simulink model "ASM_Traffic_new"  (R2024a)
settings: Solver=ode1  StartTime=SIM.tstart.v  StopTime=SIM.tend.v  FixedStep=SIM.StepSize.v  RelTol=1e-3
PostLoadFcn:
  | if any(exist('dsrtsu_mdlpostloadfcn', 'file') ~= 0), dsrtsu_mdlpostloadfcn('Execute', bdroot); end
  | try, asm_mdl_postloadfcn(bdroot, 'UpdateModel', 3600); catch, disp(lasterr); end,
InitFcn:
  | , if any(exist('rtifpga_mdlclblib', 'file') ~= 0), rtifpga_mdlclblib('Init', bdroot); end,
  | , if any(exist('dsmpb_private', 'file') ~= 0), dsmpb_private('dsmpb_mdlclblib', 'Init', bdroot); end,
undefined symbols (not defined in the file): _to_, a0b2, ASM_BrakeHydraulics_DemoSystems, ASM_VehicleDynamics_DemoSystems, b98103fe8ad365046cd0, BrakeCircuit, CPT, Crankshaft, DiscIntNeverNeededParam, dsmsi, FinalDriveAssembly, MDL, ModeSignals, Pos_BrakePedal_Maneuver, rad, RefSignals, s_to_rpm, SIM, SoftECU, Suspension, Tire, Transmission
libraries: ASM_Traffic_lib x135, simulink x100, ASM_Utils_lib x77, ASM_VehicleDynamics_lib x70, ASM_Environment_lib x22, dsmpblib x20, dsmsilib x15, MDLD_Utils_lib x10, ASM_BrakeHydraulics_lib x3
(part 12 of 63)

== system ASM_Traffic_new/Engine/Interface_Out/Control_ModelSignals ==
  State_ICEngine[0|1|2|3|4] : Inport
  n_Engine_Idle_Set[rpm] : Inport  Port=2
  Sw_Starter[0Off|1On] : Inport  Port=3
  Enable_Trq_Shift_Request[0|1] : Inport  Port=4
  Trq_Shift_Request[Nm] : Inport  Port=5
  State_StartStop[1Off|2NotReady|3Ready|4EngStopped] : Inport  Port=6
  CrankAngle_Cyl[aTDC] : Inport  Port=7
  p_Ambient[Pa] : Inport  Port=8
  T_Ambient[degC] : Inport  Port=9
  Sw_Replace_Env[0|1] : Inport  Port=10
  EngOP_Num[] : Inport  Port=11
  Pos_AccPedal_Meas[%] : Inport  Port=12
  n_Engine_Meas[rpm] : Inport  Port=13
  Trq_MeanEff_Engine_Meas[Nm] : Inport  Port=14
  Bus Creator : BusCreator  Inputs=14
  CrankAngle_Cyl[aTDC]_ : Subsystem
      mask Display: disp('')
  Enable_Trq_Shift_Request[0|1]_ : Subsystem
      mask Display: disp('')
  EngOP_Num[]_ : Subsystem
      mask Display: disp('')
  Pos_AccPedal_Meas[%]_ : Subsystem
      mask Display: disp('')
  State_ICEngine[0|1|2|3|4]_ : Subsystem
      mask Display: disp('')
  State_StartStop[1Off|2NotReady|3Ready|4EngStopped]_ : Subsystem
      mask Display: disp('')
  Sw_Replace_Env[0|1]_ : Subsystem
      mask Display: disp('')
  Sw_Starter[0Off|1On]_ : Subsystem
      mask Display: disp('')
  T_Ambient[degC]_ : Subsystem
      mask Display: disp('')
  Trq_MeanEff_Engine_Meas[Nm]_ : Subsystem
      mask Display: disp('')
  Trq_Shift_Request[Nm]_ : Subsystem
      mask Display: disp('')
  n_Engine_Idle_Set[rpm]_ : Subsystem
      mask Display: disp('')
  n_Engine_Meas[rpm]_ : Subsystem
      mask Display: disp('')
  p_Ambient[Pa]_ : Subsystem
      mask Display: disp('')
  Out : Outport  VectorParamsAs1DForOutWhenUnconnected=off
  wires:
  T_Ambient[degC]_/1(Out1) -> Bus Creator/9  "T_Ambient[degC]"
  p_Ambient[Pa]_/1(Out1) -> Bus Creator/8  "p_Ambient[Pa]"
  CrankAngle_Cyl[aTDC]_/1(Out1) -> Bus Creator/7  "CrankAngle_Cyl[aTDC]"
  T_Ambient[degC]/1 -> T_Ambient[degC]_/1(In1)
  p_Ambient[Pa]/1 -> p_Ambient[Pa]_/1(In1)
  CrankAngle_Cyl[aTDC]/1 -> CrankAngle_Cyl[aTDC]_/1(In1)
  n_Engine_Idle_Set[rpm]_/1(Out1) -> Bus Creator/2  "n_Engine_Idle_Set[rpm]"
  n_Engine_Idle_Set[rpm]/1 -> n_Engine_Idle_Set[rpm]_/1(In1)
  Bus Creator/1 -> Out/1  "Control"
  State_ICEngine[0|1|2|3|4]/1 -> State_ICEngine[0|1|2|3|4]_/1(In1)
  State_ICEngine[0|1|2|3|4]_/1(Out1) -> Bus Creator/1  "State_ICEngine[0|1|2|3|4]"
  State_StartStop[1Off|2NotReady|3Ready|4EngStopped]_/1(Out1) -> Bus Creator/6  "State_StartStop[1Off|2NotReady|3Ready|4EngStopped]"
  State_StartStop[1Off|2NotReady|3Ready|4EngStopped]/1 -> State_StartStop[1Off|2NotReady|3Ready|4EngStopped]_/1(In1)
  Trq_Shift_Request[Nm]_/1(Out1) -> Bus Creator/5  "Trq_Shift_Request[Nm]"
  Sw_Starter[0Off|1On]_/1(Out1) -> Bus Creator/3  "Sw_Starter[0Off|1On]"
  Trq_Shift_Request[Nm]/1 -> Trq_Shift_Request[Nm]_/1(In1)
  Sw_Starter[0Off|1On]/1 -> Sw_Starter[0Off|1On]_/1(In1)
  Enable_Trq_Shift_Request[0|1]_/1(Out1) -> Bus Creator/4  "Enable_Trq_Shift_Request[0|1]"
  Enable_Trq_Shift_Request[0|1]/1 -> Enable_Trq_Shift_Request[0|1]_/1(In1)
  Sw_Replace_Env[0|1]_/1(Out1) -> Bus Creator/10  "Sw_Replace_Env[0|1]"
  EngOP_Num[]/1 -> EngOP_Num[]_/1(In1)
  Trq_MeanEff_Engine_Meas[Nm]/1 -> Trq_MeanEff_Engine_Meas[Nm]_/1(In1)
  Pos_AccPedal_Meas[%]_/1(Out1) -> Bus Creator/12  "Pos_AccPedal_Meas[%]"
  EngOP_Num[]_/1(Out1) -> Bus Creator/11  "EngOP_Num[]"
  n_Engine_Meas[rpm]/1 -> n_Engine_Meas[rpm]_/1(In1)
  Pos_AccPedal_Meas[%]/1 -> Pos_AccPedal_Meas[%]_/1(In1)
  Sw_Replace_Env[0|1]/1 -> Sw_Replace_Env[0|1]_/1(In1)
  Trq_MeanEff_Engine_Meas[Nm]_/1(Out1) -> Bus Creator/14  "Trq_MeanEff_Engine_Meas[Nm]"
  n_Engine_Meas[rpm]_/1(Out1) -> Bus Creator/13  "n_Engine_Meas[rpm]"

== system ASM_Traffic_new/Engine/Interface_Out/Plant_ModelSignals ==
  Trq_MeanEff_Engine[Nm] : Inport
  Trq_Fric_Engine[Nm] : Inport  Port=2
  T_Coolant_ICE[degC] : Inport  Port=3
  Type_Engine[0Unkown|1Other|2Otto|3Diesel|4Electric] : Inport  Port=4
  Bus Creator : BusCreator  Inputs=4
  T_Coolant_ICE[degC]_ : Subsystem
      mask Display: disp('')
  Trq_Fric_Engine[Nm]_ : Subsystem
      mask Display: disp('')
  Trq_MeanEff_Engine[Nm]_ : Subsystem
      mask Display: disp('')
  Type_Engine[0Unkown|1Other|2Otto|3Diesel|4Electric]_ : Subsystem
      mask Display: disp('')
  Out : Outport  VectorParamsAs1DForOutWhenUnconnected=off
  wires:
  Trq_MeanEff_Engine[Nm]/1 -> Trq_MeanEff_Engine[Nm]_/1(In1)
  Trq_MeanEff_Engine[Nm]_/1(Out1) -> Bus Creator/1  "Trq_MeanEff_Engine[Nm]"
  Bus Creator/1 -> Out/1  "Plant"
  Trq_Fric_Engine[Nm]_/1(Out1) -> Bus Creator/2  "Trq_Fric_Engine[Nm]"
  Trq_Fric_Engine[Nm]/1 -> Trq_Fric_Engine[Nm]_/1(In1)
  T_Coolant_ICE[degC]/1 -> T_Coolant_ICE[degC]_/1(In1)
  T_Coolant_ICE[degC]_/1(Out1) -> Bus Creator/3  "T_Coolant_ICE[degC]"
  Type_Engine[0Unkown|1Other|2Otto|3Diesel|4Electric]/1 -> Type_Engine[0Unkown|1Other|2Otto|3Diesel|4Electric]_/1(In1)
  Type_Engine[0Unkown|1Other|2Otto|3Diesel|4Electric]_/1(Out1) -> Bus Creator/4  "Type_Engine[0Unkown|1Other|2Otto|3Diesel|4Electric]"

== system ASM_Traffic_new/Engine/Plant/EngineBasic ==
  note: -------------
  note: -------------
  note: Plant
  note: User Interface
  note: Inport colors:
  note: External Signals
  note: -------------
  note: Control
  note: -------------
  UserInterface : Inport
  Interface_In : Inport  Port=2
  Control : Inport  Port=3
  ASMBUS_ENGINE : GotoTagVisibility  GotoTag=ASMBUS_ENGINE
  ASMBUS_FUEL_CONSUMPTION : GotoTagVisibility  GotoTag=ASMBUS_FUEL_CONSUMPTION
  ASMSignalCollector : Subsystem
  Bus Selector1 : BusSelector  OutputSignals=Pos_AccPedal_Ctrl[%],Pos_AccPedal_Driver_Des[%],Sw_Engine_Dynamics_Fast[0|1]
  Bus Selector4 : BusSelector  OutputSignals=ExternalModel.n_Engine[rpm],ExternalModel.Reset_States[0|1]
  ENGINE : ASM_VehicleDynamics_lib/EngineBasic/ENGINE  Tag=ASM_SUBCOMPONENT  Map_Torque=MDL.EngineBasic.Engine.Map_Trq_MeanEff_Engine  Const_TimeConst_Increase=MDL.EngineBasic.Engine.Const_TimeConst_Increase  Const_TimeConst_Decrease=MDL.EngineBasic.Engine.Const_TimeConst_Decrease  Const_TimeConst_Fast=MDL.EngineBasic.Engine.Const_TimeConst_Fast  StepSize=SIM.StepSize  ASMProperties=struct('Name','ENGINE','Version','9.0','Library','ASM_VehicleDynamics_lib')  ASMInstanceName=engine  ASMInstanceID=1
  FUEL_CONSUMPTION : ASM_VehicleDynamics_lib/EngineBasic/FUEL_CONSUMPTION  Tag=ASM_SUBCOMPONENT  Const_rho_Fuel=MDL.EngineBasic.FuelConsumption.Const_rho_Fuel  Map_Specif_FuelConsumption=MDL.EngineBasic.FuelConsumption.Map_Specif_FuelConsumption  Const_Specif_Emission_CO2=MDL.EngineBasic.FuelConsumption.Const_Specif_Emission_CO2  Const_V_Displ=MDL.EngineBasic.FuelConsumption.Const_V_Displ  Const_i=MDL.EngineBasic.FuelConsumption.Const_i  Const_Q_LHV=MDL.EngineBasic.FuelConsumption.Const_Q_LHV  Const_mdot_Fuel_Idle=MDL.EngineBasic.FuelConsumption.Const_mdot_Fuel_Idle  Const_Trq_Fric_Engine_Idle=MDL.EngineBasic.FuelConsumption.Const_Trq_Fric_Engine_Idle  StepSize=SIM.StepSize  ASMProperties=struct('Name','FUEL_CONSUMPTION','Version','3.0','Library','ASM_VehicleDynamics_lib')  ASMInstanceName=fuel_consumption  ASMInstanceID=1
  ModelDesk_MC_ID_EngineBasic : ASM_Utils_lib/ModelDeskInterface/ModelDesk_MC  Tag=ASM_MAINCOMPONENT  Editable=off  MainComponent=EngineBasic
  Terminator : Terminator
  Terminator1 : Terminator
  Terminator2 : Terminator
  Terminator_4 : Terminator
  ASMSignalBus : Outport  VectorParamsAs1DForOutWhenUnconnected=off
  tag scope: ASMBUS_ENGINE=scoped, ASMBUS_FUEL_CONSUMPTION=scoped
  wires:
  FUEL_CONSUMPTION/4 -> Terminator2/1
  FUEL_CONSUMPTION/3 -> Terminator1/1
  FUEL_CONSUMPTION/2 -> Terminator/1
  FUEL_CONSUMPTION/1 -> [ASMBUS_FUEL_CONSUMPTION]
  Bus Selector1/3 -> ENGINE/4  "<Sw_Engine_Dynamics_Fast[0|1]>"
  Bus Selector1/2 -> ENGINE/3  "<Pos_AccPedal_Driver_Des[%]>"
  Bus Selector1/1 -> ENGINE/2  "<Pos_AccPedal_Ctrl[%]>"
  Interface_In/1 -> Bus Selector4/1
  ENGINE/2 -> FUEL_CONSUMPTION/1
  Control/1 -> Bus Selector1/1
  ENGINE/1 -> [ASMBUS_ENGINE]
  ASMSignalCollector/1(ASMSIgnalBus) -> ASMSignalBus/1
  Bus Selector4/1 -> FUEL_CONSUMPTION/2, ENGINE/1  "<n_Engine[rpm]>"
  Bus Selector4/2 -> FUEL_CONSUMPTION/4, ENGINE/5  "<Reset_States[0|1]>"
  UserInterface/1 -> Terminator_4/1
  ENGINE/3 -> FUEL_CONSUMPTION/3

== system ASM_Traffic_new/Engine/Plant/UserInterface ==
  note: Engine Basic
  In : Inport
  Interface_In : Inport  Port=2
  ASMSignalBus_Plant : Subsystem
  DISP_Plant : Subsystem
  PAR_Plant : Subsystem
  Out : Outport  VectorParamsAs1DForOutWhenUnconnected=off
  wires:
  Interface_In/1 -> DISP_Plant/1(Interface_In)
  PAR_Plant/1(Out) -> Out/1
  In/1 -> DISP_Plant/2(In), ASMSignalBus_Plant/1(In)

== system ASM_Traffic_new/Engine/SignalInterface/ASMSignalInterface ==
  ASMSignalBus : Inport
  Enable : EnablePort
  signal_structure : Subsystem
  wires:
  ASMSignalBus/1 -> signal_structure/1(ASMSignalBus)

== system ASM_Traffic_new/Engine/SignalInterface/ExternalOutports ==
  In1 : Inport
  Enable : EnablePort
  Engine : dsmpblib/Data Outport  Tag=ASM_MPB  Priority=-10000
      settings: SourceProductName=dSPACE Model Interface Package for Simulink (MIPS)
  Select_Outport_Signals : Subsystem
  wires:
  In1/1 -> Select_Outport_Signals/1(ASMSignalBus)
  Select_Outport_Signals/2(FuelConsumption) -> Engine/2
  Select_Outport_Signals/1(Engine) -> Engine/1

== system ASM_Traffic_new/Environment/GroundTruth/PlantModel ==
  UserInterface : Inport
  In : Inport  Port=2
  Add_Time : Subsystem
  AutomatedDrivingFunction[] : Subsystem
  Bus Creator : BusCreator  Inputs=10
  Bus Creator1 : BusCreator  Inputs=5
  Bus Selector : BusSelector  OutputSignals=Control,Info,Data
  Bus Selector1 : BusSelector  OutputSignals=Plant.Lane_Network.LaneNetwork_Data[]
  Bus Selector10 : BusSelector  OutputSignals=Plant.ManeuverScheduler.Parameters.Object_Type_ID[]
  Bus Selector11 : BusSelector  OutputSignals=Fellow_Vehicles[].Fellow_Vehicles_LightStates.High_Beam[],Fellow_Vehicles[].Fellow_Vehicles_LightStates.Reversing_Light[],Fellow_Vehicles[].Fellow_Vehicles_LightStates.Front_Fog_Light[],Fellow_Vehicles[].Fellow_Vehicles_LightStates.Head_Light[],Fellow_Vehicles[].Fellow_Vehicles_LightStates.License_Plate_Illumination[],Fellow_Vehicles[].Fellow_Vehicles_LightStates.Rear_Fog_Light[],Fellow_Vehicles[].Fellow_Vehicles_LightStates.Emergency_Veh_Illu_Fellows[],Fellow_Vehicles[].Fellow_Vehicles_LightStates.Service_Veh_Illu_Fellows[],Fellow_Vehicles[].Fellow_Vehicles_LightStates.Indicator_State[],Fellow_Vehicles[].Fellow_Vehicles_LightStates.Brake_Light[],Country_Code[]
  Bus Selector12 : BusSelector  OutputSignals=Plant.Road_TrafficFellows.Network_Item_Type_Fellows[],Plant.Road_TrafficFellows.Network_Item_Id_Fellows[],Plant.Road_TrafficFellows.LaneSection_Fellows[],Plant.Road_TrafficFellows.LaneIdx_Total_Fellows_Road[]
  Bus Selector13 : BusSelector  OutputSignals=Plant.TrafficObject_Data[]
  Bus Selector14 : BusSelector  OutputSignals=Flag_FellowUsed[0|1]
  Bus Selector{15..17,20..21} (5 alike) : BusSelector  OutputSignals=OSIGroundTruth
  Bus Selector18 : BusSelector  OutputSignals=Sensors.Plant.Sensors_Common.Sensor_Init_Ready[0Off|1On]
  Bus Selector19 : BusSelector  OutputSignals=Maneuver.Plant.ManeuverScheduler.Info.ManeuverTime[s]
  Bus Selector2 : BusSelector  OutputSignals=ExternalModel.Pos_Vehicle_CoorSys_E[x;y;z][m],ExternalModel.Angle_Vehicle_CoorSys_E[x;y;z][deg]
  Bus Selector22 : BusSelector  OutputSignals=Plant.UserSignals_Customized.GPS_Method[],Plant.UserSignals_Customized.Const_Offset_Lat[deg],Plant.UserSignals_Customized.Const_Offset_Long[deg]
  Bus Selector23 : BusSelector  OutputSignals=OSIGroundTruth.HostVehicle_Data_AutomatedDrivingFunction[]
  Bus Selector24 : BusSelector  OutputSignals=Enable_HostVehicle_Data[0Off|1On]
  Bus Selector26 : BusSelector  OutputSignals=Maneuver
  Bus Selector27 : BusSelector  OutputSignals=Interface_In
  Bus Selector{28,31,33,35} (4 alike) : BusSelector  OutputSignals=Road
  Bus Selector29 : BusSelector  OutputSignals=Maneuver
  Bus Selector3 : BusSelector  OutputSignals=Plant.Road_Info.Network_Item_Type_Veh[],Plant.Road_Info.Network_Item_Id_Veh[],Plant.Road_Info.LaneSection_Veh[],Plant.Road_ASMVeh.LaneIdx_Total_Veh_Road[]
  Bus Selector30 : BusSelector  OutputSignals=Traffic.Plant.Traffic_Signals_toEnvironment
  Bus Selector32 : BusSelector  OutputSignals=Traffic.Plant.ObjectParameters
  Bus Selector34 : BusSelector  OutputSignals=Road.UserInterface.Objects_DataStreams[]
  Bus Selector4 : BusSelector  OutputSignals=Plant.ManeuverScheduler.Info.ManeuverState[],Plant.ManeuverScheduler.Info.ManeuverTime[s]
  Bus Selector5 : BusSelector  OutputSignals=FellowParameters.TrafficObject_Type_Fellows[],TrafficObjects.TrafficObject_Type_Data[]
  Bus Selector6 : BusSelector  OutputSignals=OSIGroundTruth.TrafficLight_Counter[]
  Bus Selector7 : BusSelector  OutputSignals=Ego_Vehicle[].Ego_Vehicle_ID[],Ego_Vehicle[].Ego_Vehicle_Driver_ID[]
  Bus Selector8 : BusSelector  OutputSignals=Ego_Vehicle[].Ego_Vehicle_LightStates[]
  Bus Selector9 : BusSelector  OutputSignals=OSIGroundTruth.Environmental_Conditions[]
  GetFellowPositionVector : Subsystem
  GroundTruth_Data_Access : Subsystem
  HostVehicle_Data_Access : Subsystem
  Length_GT_Area_Lat_Ext : Constant  Value=[20;20]
  Length_GT_Area_Long_Ext : Constant  Value=[100;50]
  Mux1 : Mux  Inputs=3
  OSI_GROUNDTRUTH_INTERFACE : ASM_Traffic_lib/GroundTruth/OSI_GROUNDTRUTH_INTERFACE  Tag=ASM_SUBCOMPONENT  Sw_Interface_Mode=MDL.Traffic.GroundTruth.OSIInterface.Sw_Interface_Mode  Sw_GT_Area_Definition_Mode=MDL.Traffic.GroundTruth.OSIInterface.Sw_GT_Area_Definition_Mode  Const_Length_GT_Area_Front=MDL.Traffic.GroundTruth.OSIInterface.Const_Length_GT_Area_Front  Const_Length_GT_Area_Rear=MDL.Traffic.GroundTruth.OSIInterface.Const_Length_GT_Area_Rear  Const_Length_GT_Area_Left=MDL.Traffic.GroundTruth.OSIInterface.Const_Length_GT_Area_Left  Const_Length_GT_Area_Right=MDL.Traffic.GroundTruth.OSIInterface.Const_Length_GT_Area_Right  Sw_Quadrant_Def_Mode=MDL.Traffic.GroundTruth.OSIInterface.Sw_Quadrant_Def_Mode  Const_Quad_Dim_x=MDL.Traffic.GroundTruth.OSIInterface.Const_Quad_Dim_x  Const_Quad_Dim_y=MDL.Traffic.GroundTruth.OSIInterface.Const_Quad_Dim_y  Const_Max_Num_LB_In_GT_Area=MDL.Traffic.GroundTruth.OSIInterface.Const_Max_Num_LB_In_GT_Area  Const_Max_Num_Points_Per_LB=MDL.Traffic.GroundTruth.OSIInterface.Const_Max_Num_Points_Per_LB  Const_Max_Num_Lanes_In_GT_Area=MDL.Traffic.GroundTruth.OSIInterface.Const_Max_Num_Lanes_In_GT_Area  Const_Max_Num_Lane_Pairings_Per_Lane=MDL.Traffic.GroundTruth.OSIInterface.Const_Max_Num_Lane_Pairings_Per_Lane  Const_Max_Num_Free_LB_Per_Lane=MDL.Traffic.GroundTruth.OSIInterface.Const_Max_Num_Free_LB_Per_Lane  Const_Max_Num_PolyPts_Per_Object=MDL.Traffic.GroundTruth.OSIInterface.Const_Max_Num_PolyPts_Per_Object  StepSize=SIM.StepSize  ASMProperties=struct('Name','OSI_GROUNDTRUTH_INTERFACE','Version','10.0','Library','ASM_Traffic_lib')  ASMInstanceName=osi_groundtruth_interface  ASMInstanceID=1
  ObjectDataStreams : Subsystem
  Running_Maneuver : Subsystem
  Signal Specification{1..15} (15 alike) : SignalSpecification  Dimensions=MDL.Traffic.MaxNumFellows.v
  Terminator : Terminator
  TrafficLight_Counter : Subsystem
  VehicleBasics : Subsystem
  VehicleBrakeSystem : Subsystem
  VehicleLocalization : Subsystem
  VehiclePowertrain : Subsystem
  VehicleSteering : Subsystem
  VehicleWheels : Subsystem
  ASMSignalBus : Outport  VectorParamsAs1DForOutWhenUnconnected=off
  wires:
  Bus Selector23/1 -> AutomatedDrivingFunction[]/1(In)  "<HostVehicle_Data_AutomatedDrivingFunction[]>"
  In/1 -> Bus Selector18/1, Bus Selector26/1, Bus Selector27/1, Bus Selector28/1, Bus Selector30/1, Bus Selector29/1, Bus Selector31/1, Bus Selector33/1, Bus Selector34/1, Bus Selector35/1, VehiclePowertrain/1(In), VehicleBasics/1(In), VehicleWheels/1(In), VehicleBrakeSystem/1(In), VehicleSteering/1(In), VehicleLocalization/1(In), Bus Selector19/1, Bus Selector32/1
  Bus Selector21/1 -> VehicleWheels/2(OSIGroundTruth), VehicleBasics/2(OSIGroundTruth)  "<OSIGroundTruth>"
  GroundTruth_Data_Access/11(MovingObject[]) -> Bus Creator1/5  "OpenSimulationInterface"
  Bus Selector/3 -> Bus Creator1/3  "<Data>"
  Bus Selector/1 -> Bus Creator1/1  "<Control>"
  Bus Selector/2 -> Bus Creator1/2  "<Info>"
  Bus Creator1/1 -> ASMSignalBus/1  "Plant"
  Bus Creator/1 -> Bus Creator1/4  "Data_Access"
  Bus Selector19/1 -> Add_Time/1(TimeSignal[s])  "<ManeuverTime[s]>"
  Add_Time/1(EnvironmentConditions_Out[]) -> OSI_GROUNDTRUTH_INTERFACE/33
  Bus Selector18/1 -> OSI_GROUNDTRUTH_INTERFACE/1  "<Sensor_Init_Ready[0Off|1On]>"
  Bus Selector29/1 -> Bus Selector10/1  "<Maneuver>"
  Bus Selector35/1 -> Bus Selector22/1  "<Road>"
  Bus Selector33/1 -> Bus Selector13/1, Bus Selector1/1  "<Road>"
  Bus Selector31/1 -> Bus Selector12/1  "<Road>"
  Bus Selector17/1 -> Bus Selector11/1  "<OSIGroundTruth>"
  Bus Selector16/1 -> Bus Selector8/1  "<OSIGroundTruth>"
  Bus Selector15/1 -> Bus Selector7/1  "<OSIGroundTruth>"
  OSI_GROUNDTRUTH_INTERFACE/1 -> Bus Selector/1  "Interface"
  Signal Specification15/1 -> OSI_GROUNDTRUTH_INTERFACE/31
  Signal Specification14/1 -> OSI_GROUNDTRUTH_INTERFACE/30
  Signal Specification13/1 -> OSI_GROUNDTRUTH_INTERFACE/29
  Signal Specification12/1 -> OSI_GROUNDTRUTH_INTERFACE/28
  Signal Specification6/1 -> OSI_GROUNDTRUTH_INTERFACE/27
  Signal Specification5/1 -> OSI_GROUNDTRUTH_INTERFACE/26
  Signal Specification4/1 -> OSI_GROUNDTRUTH_INTERFACE/25
  Signal Specification3/1 -> OSI_GROUNDTRUTH_INTERFACE/24
  Signal Specification2/1 -> OSI_GROUNDTRUTH_INTERFACE/23
  Signal Specification1/1 -> OSI_GROUNDTRUTH_INTERFACE/22
  Bus Selector2/2 -> OSI_GROUNDTRUTH_INTERFACE/7  "<Angle_Vehicle_CoorSys_E[x;y;z][deg]>"
  Bus Selector2/1 -> OSI_GROUNDTRUTH_INTERFACE/6  "<Pos_Vehicle_CoorSys_E[x;y;z][m]>"
  Length_GT_Area_Long_Ext/1 -> OSI_GROUNDTRUTH_INTERFACE/37
  OSI_GROUNDTRUTH_INTERFACE/2 -> Terminator/1
  Bus Selector22/3 -> Mux1/3  "<Const_Offset_Long[deg]>"
  Bus Selector22/2 -> Mux1/2  "<Const_Offset_Lat[deg]>"
  Bus Selector22/1 -> Mux1/1  "<GPS_Method[]>"
  Mux1/1 -> OSI_GROUNDTRUTH_INTERFACE/41
  TrafficLight_Counter/1(TrafficLight_Counter[]) -> OSI_GROUNDTRUTH_INTERFACE/40
  Bus Selector11/7 -> Signal Specification12/1  "<Emergency_Veh_Illu_Fellows[]>"
  Bus Selector11/8 -> Signal Specification13/1  "<Service_Veh_Illu_Fellows[]>"
  OSI_GROUNDTRUTH_INTERFACE/3 -> GroundTruth_Data_Access/1(OSI_GT_Data)
  Bus Selector5/1 -> OSI_GROUNDTRUTH_INTERFACE/21  "<TrafficObject_Type_Fellows[]>"
  Bus Selector5/2 -> OSI_GROUNDTRUTH_INTERFACE/35  "<TrafficObject_Type_Data[]>"
  Bus Selector4/2 -> OSI_GROUNDTRUTH_INTERFACE/3  "<ManeuverTime[s]>"
  Bus Selector10/1 -> OSI_GROUNDTRUTH_INTERFACE/12  "<Object_Type_ID[]>"
  Bus Selector7/1 -> OSI_GROUNDTRUTH_INTERFACE/4  "<Ego_Vehicle_ID[]>"
  Bus Selector7/2 -> OSI_GROUNDTRUTH_INTERFACE/5  "<Ego_Vehicle_Driver_ID[]>"
  Bus Selector8/1 -> OSI_GROUNDTRUTH_INTERFACE/13  "<Ego_Vehicle_LightStates[]>"
  Bus Selector3/1 -> OSI_GROUNDTRUTH_INTERFACE/8  "<Network_Item_Type_Veh[]>"
  Bus Selector3/2 -> OSI_GROUNDTRUTH_INTERFACE/9  "<Network_Item_Id_Veh[]>"
  Bus Selector3/3 -> OSI_GROUNDTRUTH_INTERFACE/10  "<LaneSection_Veh[]>"
  Bus Selector3/4 -> OSI_GROUNDTRUTH_INTERFACE/11  "<LaneIdx_Total_Veh_Road[]>"
  Bus Selector11/1 -> Signal Specification1/1  "<High_Beam[]>"
  Bus Selector11/2 -> Signal Specification2/1  "<Reversing_Light[]>"
  Bus Selector11/3 -> Signal Specification3/1  "<Front_Fog_Light[]>"
  Bus Selector11/4 -> Signal Specification4/1  "<Head_Light[]>"
  Bus Selector11/5 -> Signal Specification5/1  "<License_Plate_Illumination[]>"
  Bus Selector11/6 -> Signal Specification6/1  "<Rear_Fog_Light[]>"
  Bus Selector11/9 -> Signal Specification14/1  "<Indicator_State[]>"
  Bus Selector11/10 -> Signal Specification15/1  "<Brake_Light[]>"
  Bus Selector11/11 -> OSI_GROUNDTRUTH_INTERFACE/32  "<Country_Code[]>"
  Bus Selector9/1 -> Add_Time/2(Environmental_Conditions[])  "<Environmental_Conditions[]>"
  UserInterface/1 -> Bus Selector15/1, Bus Selector16/1, Bus Selector17/1, Bus Selector9/1, Bus Selector6/1, Bus Selector23/1, Bus Selector21/1, Bus Selector20/1
  Bus Selector14/1 -> Signal Specification7/1  "<Flag_FellowUsed[0|1]>"
  GetFellowPositionVector/2(Angle_Fellows[deg]) -> OSI_GROUNDTRUTH_INTERFACE/16
  Signal Specification7/1 -> OSI_GROUNDTRUTH_INTERFACE/14
  Signal Specification10/1 -> OSI_GROUNDTRUTH_INTERFACE/18
  Signal Specification11/1 -> OSI_GROUNDTRUTH_INTERFACE/19
  Signal Specification8/1 -> OSI_GROUNDTRUTH_INTERFACE/20
  Signal Specification9/1 -> OSI_GROUNDTRUTH_INTERFACE/17
  Bus Selector12/1 -> Signal Specification9/1  "<Network_Item_Type_Fellows[]>"
  Bus Selector12/2 -> Signal Specification10/1  "<Network_Item_Id_Fellows[]>"
  Bus Selector12/3 -> Signal Specification11/1  "<LaneSection_Fellows[]>"
  Bus Selector12/4 -> Signal Specification8/1  "<LaneIdx_Total_Fellows_Road[]>"
  Bus Selector1/1 -> OSI_GROUNDTRUTH_INTERFACE/36  "<LaneNetwork_Data[]>"
  Bus Selector13/1 -> OSI_GROUNDTRUTH_INTERFACE/34  "<TrafficObject_Data[]>"
  GroundTruth_Data_Access/10(Num_TrfSigns_in_GT_Area[]) -> Bus Creator/10  "Num_TrfSigns_in_GT_Area[]"
  GroundTruth_Data_Access/9(Num_TrfSigns[]) -> Bus Creator/9  "Num_TrfSigns[]"
  GroundTruth_Data_Access/8(Num_TrfLights_in_GT_Area[]) -> Bus Creator/8  "Num_TrfLights_in_GT_Area[]"
  GroundTruth_Data_Access/7(Num_TrfLights[]) -> Bus Creator/7  "Num_TrfLights[]"
  GroundTruth_Data_Access/6(Num_Lanes[]) -> Bus Creator/6  "Num_Lanes[]"
  GroundTruth_Data_Access/5(Num_Laneboundaries[]) -> Bus Creator/5  "Num_Laneboundaries[]"
  GroundTruth_Data_Access/4(Num_StatObj_in_GT_Area[]) -> Bus Creator/4  "Num_StatObj_in_GT_Area[]"
  GroundTruth_Data_Access/3(Num_StatObj[]) -> Bus Creator/3  "Num_StatObj[]"
  GroundTruth_Data_Access/2(Num_MovObj_in_GT_Area[]) -> Bus Creator/2  "Num_MovObj_in_GT_Area[]"
  GroundTruth_Data_Access/1(Num_MovObj[]) -> Bus Creator/1  "Num_MovObj[]"
  Length_GT_Area_Lat_Ext/1 -> OSI_GROUNDTRUTH_INTERFACE/38
  Bus Selector4/1 -> Running_Maneuver/1(ManeuverState[])  "<ManeuverState[]>"
  Running_Maneuver/1(EnableRun[0Off|1On]) -> OSI_GROUNDTRUTH_INTERFACE/2
  ObjectDataStreams/1(Objects_DataStreams[]) -> OSI_GROUNDTRUTH_INTERFACE/39
  Bus Selector6/1 -> TrafficLight_Counter/1(In)  "<TrafficLight_Counter[]>"
  GetFellowPositionVector/1(Pos_Fellows_MainPnt_CoorSys_E[x;y;z][m]) -> OSI_GROUNDTRUTH_INTERFACE/15  "Pos_Fellows_MainPnt_CoorSys_E[x;y;z][m]"
  Bus Selector26/1 -> Bus Selector4/1  "<Maneuver>"
  Bus Selector28/1 -> Bus Selector3/1  "<Road>"
  Bus Selector30/1 -> Bus Selector14/1, GetFellowPositionVector/1(FellowPositions)  "<Traffic_Signals_toEnvironment>"
  Bus Selector27/1 -> Bus Selector2/1  "<Interface_In>"
  Bus Selector32/1 -> Bus Selector5/1  "<ObjectParameters>"
  Bus Selector34/1 -> ObjectDataStreams/1(In)  "<Objects_DataStreams[]>"
  VehiclePowertrain/2(Pos_ClutchPedal[0_1]) -> OSI_GROUNDTRUTH_INTERFACE/49
  VehiclePowertrain/3(Gear[]) -> OSI_GROUNDTRUTH_INTERFACE/50
  VehiclePowertrain/4(n_Engine[rpm]) -> OSI_GROUNDTRUTH_INTERFACE/51
  VehiclePowertrain/5(Type_Engine[0Unkown|1Other|2Otto|3Diesel|4Electric]) -> OSI_GROUNDTRUTH_INTERFACE/52
  VehiclePowertrain/6(Trq_Engine[Nm]) -> OSI_GROUNDTRUTH_INTERFACE/53
  VehicleWheels/4(Slip_x_Wheel[]) -> OSI_GROUNDTRUTH_INTERFACE/57
  VehicleWheels/3(omega_Wheel[rad|s]) -> OSI_GROUNDTRUTH_INTERFACE/56
  VehicleWheels/2(Wheel_Idx[]) -> OSI_GROUNDTRUTH_INTERFACE/55
  VehicleWheels/1(Axle_Idx[]) -> OSI_GROUNDTRUTH_INTERFACE/54
  VehicleBasics/2(OperatingState[]) -> OSI_GROUNDTRUTH_INTERFACE/59
  VehicleBasics/1(m_TotalVehicle[kg]) -> OSI_GROUNDTRUTH_INTERFACE/58
  AutomatedDrivingFunction[]/1(AutomatedDrivingFunction[]) -> OSI_GROUNDTRUTH_INTERFACE/60
  VehicleSteering/2(Angle_SteeringWheel_dt_SteeringSystem[rad|s]) -> OSI_GROUNDTRUTH_INTERFACE/44
  VehicleSteering/1(Angle_SteeringWheel_SteeringSystem[rad]) -> OSI_GROUNDTRUTH_INTERFACE/43
  VehicleSteering/3(Trq_SteeringWheel_SteeringSystem[Nm]) -> OSI_GROUNDTRUTH_INTERFACE/45
  VehiclePowertrain/1(Pos_AccPedal[0_1]) -> OSI_GROUNDTRUTH_INTERFACE/48
  VehicleBrakeSystem/1(Pos_BrakePedal[0_1]) -> OSI_GROUNDTRUTH_INTERFACE/46
  VehicleLocalization/1(Pos_Veh_BoundingBox_GPS[Long;Lat;Alt][deg;deg;m]) -> OSI_GROUNDTRUTH_INTERFACE/47
  OSI_GROUNDTRUTH_INTERFACE/4 -> HostVehicle_Data_Access/1(OSI_HV_Data)  "HostVehicle_Data[]"
  Bus Selector20/1 -> Bus Selector24/1  "<OSIGroundTruth>"
  Bus Selector24/1 -> OSI_GROUNDTRUTH_INTERFACE/42  "<Enable_HostVehicle_Data[0Off|1On]>"

== system ASM_Traffic_new/Environment/GroundTruth/UserInterface ==
  note: GroundTruth
  Interface_In : Inport
  In : Inport  Port=2
  ASMSignalBus_Plant : Subsystem
  DISP_Plant : Subsystem
  PAR_Plant : Subsystem
  Out : Outport  VectorParamsAs1DForOutWhenUnconnected=off
  wires:
  PAR_Plant/1(Out) -> Out/1
  In/1 -> ASMSignalBus_Plant/1(In), PAR_Plant/2(In), DISP_Plant/1(In)
  Interface_In/1 -> PAR_Plant/1(Interface_In)

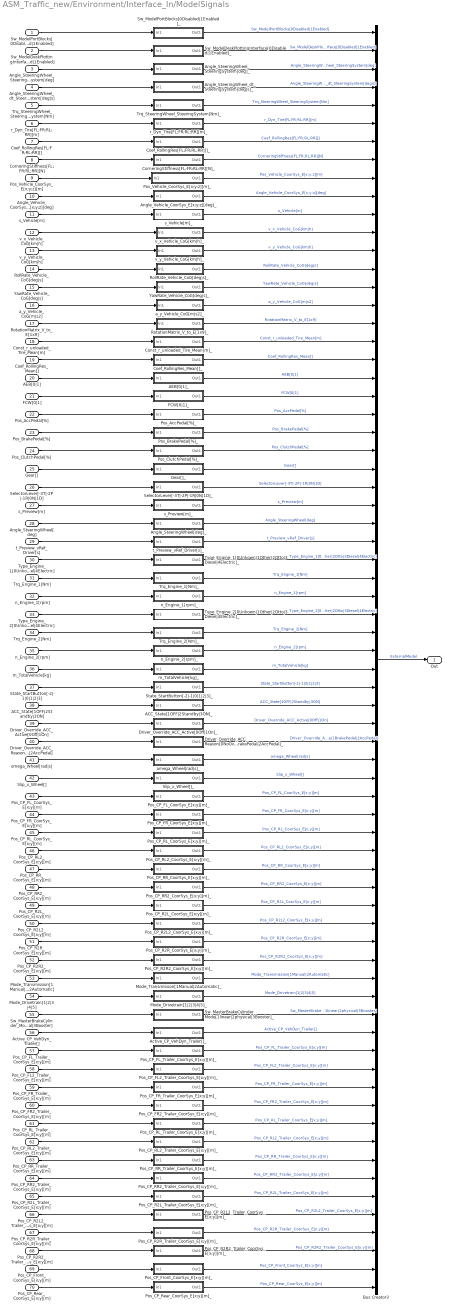
== system ASM_Traffic_new/Environment/Interface_In/ModelSignals ==
  Sw_ModelPortBlocks[0Disabled|1Enabled] : Inport
  Sw_ModelDeskPlottingInterface[0Disabled|1Enabled] : Inport  Port=2
  Angle_SteeringWheel_SteeringSystem[deg] : Inport  Port=3
  Angle_SteeringWheel_dt_SteeringSystem[deg|s] : Inport  Port=4
  Trq_SteeringWheel_SteeringSystem[Nm] : Inport  Port=5
  r_Dyn_Tire[FL;FR;RL;RR][m] : Inport  Port=6
  Coef_RollingRes[FL;FR;RL;RR][] : Inport  Port=7
  CorneringStiffness[FL;FR;RL;RR][N] : Inport  Port=8
  Pos_Vehicle_CoorSys_E[x;y;z][m] : Inport  Port=9
  Angle_Vehicle_CoorSys_E[x;y;z][deg] : Inport  Port=10
  s_Vehicle[m] : Inport  Port=11
  v_x_Vehicle_CoG[km|h] : Inport  Port=12
  v_y_Vehicle_CoG[km|h] : Inport  Port=13
  RollRate_Vehicle_CoG[deg|s] : Inport  Port=14
  YawRate_Vehicle_CoG[deg|s] : Inport  Port=15
  a_y_Vehicle_CoG[m|s2] : Inport  Port=16
  RotationMatrix_V_to_E[1x9] : Inport  Port=17
  Const_r_unloaded_Tire_Mean[m] : Inport  Port=18
  Coef_RollingRes_Mean[] : Inport  Port=19
  AEB[0|1] : Inport  Port=20
  FCW[0|1] : Inport  Port=21
  Pos_AccPedal[%] : Inport  Port=22
  Pos_BrakePedal[%] : Inport  Port=23
  Pos_ClutchPedal[%] : Inport  Port=24
  Gear[] : Inport  Port=25
  SelectorLever[-3T|-2P|-1R|0N|1D] : Inport  Port=26
  s_Preview[m] : Inport  Port=27
  Angle_SteeringWheel[deg] : Inport  Port=28
  t_Preview_vRef_Driver[s] : Inport  Port=29
  Type_Engine_1[0Unkown|1Other|2Otto|3Diesel|4Electric] : Inport  Port=30
  Trq_Engine_1[Nm] : Inport  Port=31
  n_Engine_1[rpm] : Inport  Port=32
  Type_Engine_2[0Unkown|1Other|2Otto|3Diesel|4Electric] : Inport  Port=33
  Trq_Engine_2[Nm] : Inport  Port=34
  n_Engine_2[rpm] : Inport  Port=35
  m_TotalVehicle[kg] : Inport  Port=36
  State_StartButton[-2|-1|0|1|2|3] : Inport  Port=37
  ACC_State[1OFF|2Standby|3ON] : Inport  Port=38
  Driver_Override_ACC_Active[0Off|1On] : Inport  Port=39
  Driver_Override_ACC_Reason[0NoOverride|1BrakePedal|2AccPedal] : Inport  Port=40
  omega_Wheel[rad|s] : Inport  Port=41
  Slip_x_Wheel[] : Inport  Port=42
  Pos_CP_FL_CoorSys_E[x;y][m] : Inport  Port=43
  Pos_CP_FR_CoorSys_E[x;y][m] : Inport  Port=44
  Pos_CP_RL_CoorSys_E[x;y][m] : Inport  Port=45
  Pos_CP_RL2_CoorSys_E[x;y][m] : Inport  Port=46
  Pos_CP_RR_CoorSys_E[x;y][m] : Inport  Port=47
  Pos_CP_RR2_CoorSys_E[x;y][m] : Inport  Port=48
  Pos_CP_R2L_CoorSys_E[x;y][m] : Inport  Port=49
  Pos_CP_R2L2_CoorSys_E[x;y][m] : Inport  Port=50
  Pos_CP_R2R_CoorSys_E[x;y][m] : Inport  Port=51
  Pos_CP_R2R2_CoorSys_E[x;y][m] : Inport  Port=52
  Mode_Transmission[1Manual|2Automatic] : Inport  Port=53
  Mode_Drivetrain[1|2|3|4|5] : Inport  Port=54
  Sw_MasterBrakeCylinder_Mode[1linear|2physical|3Booster] : Inport  Port=55
  Active_CP_VehDyn_Trailer[] : Inport  Port=56
  Pos_CP_FL_Trailer_CoorSys_E[x;y][m] : Inport  Port=57
  Pos_CP_FL2_Trailer_CoorSys_E[x;y][m] : Inport  Port=58
  Pos_CP_FR_Trailer_CoorSys_E[x;y][m] : Inport  Port=59
  Pos_CP_FR2_Trailer_CoorSys_E[x;y][m] : Inport  Port=60
  Pos_CP_RL_Trailer_CoorSys_E[x;y][m] : Inport  Port=61
  Pos_CP_RL2_Trailer_CoorSys_E[x;y][m] : Inport  Port=62
  Pos_CP_RR_Trailer_CoorSys_E[x;y][m] : Inport  Port=63
  Pos_CP_RR2_Trailer_CoorSys_E[x;y][m] : Inport  Port=64
  Pos_CP_R2L_Trailer_CoorSys_E[x;y][m] : Inport  Port=65
  Pos_CP_R2L2_Trailer_CoorSys_E[x;y][m] : Inport  Port=66
  Pos_CP_R2R_Trailer_CoorSys_E[x;y][m] : Inport  Port=67
  Pos_CP_R2R2_Trailer_CoorSys_E[x;y][m] : Inport  Port=68
  Pos_CP_Front_CoorSys_E[x;y][m] : Inport  Port=69
  Pos_CP_Rear_CoorSys_E[x;y][m] : Inport  Port=70
  ACC_State[1OFF|2Standby|3ON]_ : Subsystem
      mask Display: disp('')
  AEB[0|1]_ : Subsystem
      mask Display: disp('')
  Active_CP_VehDyn_Trailer[]_ : Subsystem
      mask Display: disp('')
  Angle_SteeringWheel[deg]_ : Subsystem
      mask Display: disp('')
  Angle_SteeringWheel_SteeringSystem[deg]_ : Subsystem
      mask Display: disp('')
  Angle_SteeringWheel_dt_SteeringSystem[deg|s]_ : Subsystem
      mask Display: disp('')
  Angle_Vehicle_CoorSys_E[x;y;z][deg]_ : Subsystem
      mask Display: disp('')
  Bus Creator3 : BusCreator  Inputs=70
  Coef_RollingRes[FL;FR;RL;RR][]_ : Subsystem
      mask Display: disp('')
  Coef_RollingRes_Mean[]_ : Subsystem
      mask Display: disp('')
  Const_r_unloaded_Tire_Mean[m]_ : Subsystem
      mask Display: disp('')
  CorneringStiffness[FL;FR;RL;RR][N]_ : Subsystem
      mask Display: disp('')
  Driver_Override_ACC_Active[0Off|1On]_ : Subsystem
      mask Display: disp('')
  Driver_Override_ACC_Reason[0NoOverride|1BrakePedal|2AccPedal]_ : Subsystem
      mask Display: disp('')
  FCW[0|1]_ : Subsystem
      mask Display: disp('')
  Gear[]_ : Subsystem
      mask Display: disp('')
  Mode_Drivetrain[1|2|3|4|5]_ : Subsystem
      mask Display: disp('')
  Mode_Transmission[1Manual|2Automatic]_ : Subsystem
      mask Display: disp('')
  Pos_AccPedal[%]_ : Subsystem
      mask Display: disp('')
  Pos_BrakePedal[%]_ : Subsystem
      mask Display: disp('')
  Pos_CP_FL2_Trailer_CoorSys_E[x;y][m]_ : Subsystem
      mask Display: disp('')
  Pos_CP_FL_CoorSys_E[x;y][m]_ : Subsystem
      mask Display: disp('')
  Pos_CP_FL_Trailer_CoorSys_E[x;y][m]_ : Subsystem
      mask Display: disp('')
  Pos_CP_FR2_Trailer_CoorSys_E[x;y][m]_ : Subsystem
      mask Display: disp('')
  Pos_CP_FR_CoorSys_E[x;y][m]_ : Subsystem
      mask Display: disp('')
  Pos_CP_FR_Trailer_CoorSys_E[x;y][m]_ : Subsystem
      mask Display: disp('')
  Pos_CP_Front_CoorSys_E[x;y][m]_ : Subsystem
      mask Display: disp('')
  Pos_CP_R2L2_CoorSys_E[x;y][m]_ : Subsystem
      mask Display: disp('')
  Pos_CP_R2L2_Trailer_CoorSys_E[x;y][m]_ : Subsystem
      mask Display: disp('')
  Pos_CP_R2L_CoorSys_E[x;y][m]_ : Subsystem
      mask Display: disp('')
  Pos_CP_R2L_Trailer_CoorSys_E[x;y][m]_ : Subsystem
      mask Display: disp('')
  Pos_CP_R2R2_CoorSys_E[x;y][m]_ : Subsystem
      mask Display: disp('')
  Pos_CP_R2R2_Trailer_CoorSys_E[x;y][m]_ : Subsystem
      mask Display: disp('')
  Pos_CP_R2R_CoorSys_E[x;y][m]_ : Subsystem
      mask Display: disp('')
  Pos_CP_R2R_Trailer_CoorSys_E[x;y][m]_ : Subsystem
      mask Display: disp('')
  Pos_CP_RL2_CoorSys_E[x;y][m]_ : Subsystem
      mask Display: disp('')
  Pos_CP_RL2_Trailer_CoorSys_E[x;y][m]_ : Subsystem
      mask Display: disp('')
  Pos_CP_RL_CoorSys_E[x;y][m]_ : Subsystem
      mask Display: disp('')
  Pos_CP_RL_Trailer_CoorSys_E[x;y][m]_ : Subsystem
      mask Display: disp('')
  Pos_CP_RR2_CoorSys_E[x;y][m]_ : Subsystem
      mask Display: disp('')
  Pos_CP_RR2_Trailer_CoorSys_E[x;y][m]_ : Subsystem
      mask Display: disp('')
  Pos_CP_RR_CoorSys_E[x;y][m]_ : Subsystem
      mask Display: disp('')
  Pos_CP_RR_Trailer_CoorSys_E[x;y][m]_ : Subsystem
      mask Display: disp('')
  Pos_CP_Rear_CoorSys_E[x;y][m]_ : Subsystem
      mask Display: disp('')
  Pos_ClutchPedal[%]_ : Subsystem
      mask Display: disp('')
  Pos_Vehicle_CoorSys_E[x;y;z][m]_ : Subsystem
      mask Display: disp('')
  RollRate_Vehicle_CoG[deg|s]_ : Subsystem
      mask Display: disp('')
  RotationMatrix_V_to_E[1x9]_ : Subsystem
      mask Display: disp('')
  SelectorLever[-3T|-2P|-1R|0N|1D]_ : Subsystem
      mask Display: disp('')
  Slip_x_Wheel[]_ : Subsystem
      mask Display: disp('')
  State_StartButton[-2|-1|0|1|2|3]_ : Subsystem
      mask Display: disp('')
  Sw_MasterBrakeCylinder_Mode[1linear|2physical|3Booster]_ : Subsystem
      mask Display: disp('')
  Sw_ModelDeskPlottingInterface[0Disabled|1Enabled]_ : Subsystem
  Sw_ModelPortBlocks[0Disabled|1Enabled]_ : Subsystem
  Trq_Engine_1[Nm]_ : Subsystem
      mask Display: disp('')
  Trq_Engine_2[Nm]_ : Subsystem
      mask Display: disp('')
  Trq_SteeringWheel_SteeringSystem[Nm]_ : Subsystem
      mask Display: disp('')
  Type_Engine_1[0Unkown|1Other|2Otto|3Diesel|4Electric]_ : Subsystem
      mask Display: disp('')
  Type_Engine_2[0Unkown|1Other|2Otto|3Diesel|4Electric]_ : Subsystem
      mask Display: disp('')
  YawRate_Vehicle_CoG[deg|s]_ : Subsystem
      mask Display: disp('')
  a_y_Vehicle_CoG[m|s2]_ : Subsystem
      mask Display: disp('')
  m_TotalVehicle[kg]_ : Subsystem
      mask Display: disp('')
  n_Engine_1[rpm]_ : Subsystem
      mask Display: disp('')
  n_Engine_2[rpm]_ : Subsystem
      mask Display: disp('')
  omega_Wheel[rad|s]_ : Subsystem
      mask Display: disp('')
  r_Dyn_Tire[FL;FR;RL;RR][m]_ : Subsystem
      mask Display: disp('')
  s_Preview[m]_ : Subsystem
      mask Display: disp('')
  s_Vehicle[m]_ : Subsystem
      mask Display: disp('')
  t_Preview_vRef_Driver[s]_ : Subsystem
      mask Display: disp('')
  v_x_Vehicle_CoG[km|h]_ : Subsystem
      mask Display: disp('')
  v_y_Vehicle_CoG[km|h]_ : Subsystem
      mask Display: disp('')
  Out : Outport  VectorParamsAs1DForOutWhenUnconnected=off
  wires:
  Pos_CP_Front_CoorSys_E[x;y][m]/1 -> Pos_CP_Front_CoorSys_E[x;y][m]_/1(In1)
  Pos_CP_Rear_CoorSys_E[x;y][m]_/1(Out1) -> Bus Creator3/70  "Pos_CP_Rear_CoorSys_E[x;y][m]"
  Pos_CP_Rear_CoorSys_E[x;y][m]/1 -> Pos_CP_Rear_CoorSys_E[x;y][m]_/1(In1)
  Pos_CP_Front_CoorSys_E[x;y][m]_/1(Out1) -> Bus Creator3/69  "Pos_CP_Front_CoorSys_E[x;y][m]"
  Sw_ModelDeskPlottingInterface[0Disabled|1Enabled]_/1(Out1) -> Bus Creator3/2  "Sw_ModelDeskPlottingInterface[0Disabled|1Enabled]"
  Sw_ModelPortBlocks[0Disabled|1Enabled]_/1(Out1) -> Bus Creator3/1  "Sw_ModelPortBlocks[0Disabled|1Enabled]"
  Sw_ModelDeskPlottingInterface[0Disabled|1Enabled]/1 -> Sw_ModelDeskPlottingInterface[0Disabled|1Enabled]_/1(In1)
  Sw_ModelPortBlocks[0Disabled|1Enabled]/1 -> Sw_ModelPortBlocks[0Disabled|1Enabled]_/1(In1)
  Bus Creator3/1 -> Out/1  "ExternalModel"
  Trq_SteeringWheel_SteeringSystem[Nm]/1 -> Trq_SteeringWheel_SteeringSystem[Nm]_/1(In1)
  Angle_SteeringWheel_SteeringSystem[deg]/1 -> Angle_SteeringWheel_SteeringSystem[deg]_/1(In1)
  Angle_SteeringWheel_SteeringSystem[deg]_/1(Out1) -> Bus Creator3/3  "Angle_SteeringWheel_SteeringSystem[deg]"
  Trq_SteeringWheel_SteeringSystem[Nm]_/1(Out1) -> Bus Creator3/5  "Trq_SteeringWheel_SteeringSystem[Nm]"
  Pos_CP_RR2_CoorSys_E[x;y][m]_/1(Out1) -> Bus Creator3/48  "Pos_CP_RR2_CoorSys_E[x;y][m]"
  Coef_RollingRes[FL;FR;RL;RR][]_/1(Out1) -> Bus Creator3/7  "Coef_RollingRes[FL;FR;RL;RR][]"
  Coef_RollingRes_Mean[]_/1(Out1) -> Bus Creator3/19  "Coef_RollingRes_Mean[]"
  Active_CP_VehDyn_Trailer[]_/1(Out1) -> Bus Creator3/56  "Active_CP_VehDyn_Trailer[]"
  Pos_CP_RR_Trailer_CoorSys_E[x;y][m]_/1(Out1) -> Bus Creator3/63  "Pos_CP_RR_Trailer_CoorSys_E[x;y][m]"
  Pos_CP_FL_Trailer_CoorSys_E[x;y][m]_/1(Out1) -> Bus Creator3/57  "Pos_CP_FL_Trailer_CoorSys_E[x;y][m]"
  Pos_CP_R2R_CoorSys_E[x;y][m]_/1(Out1) -> Bus Creator3/51  "Pos_CP_R2R_CoorSys_E[x;y][m]"
  Pos_CP_R2R2_Trailer_CoorSys_E[x;y][m]_/1(Out1) -> Bus Creator3/68  "Pos_CP_R2R2_Trailer_CoorSys_E[x;y][m]"
  Pos_CP_R2L_Trailer_CoorSys_E[x;y][m]_/1(Out1) -> Bus Creator3/65  "Pos_CP_R2L_Trailer_CoorSys_E[x;y][m]"
  Pos_CP_FR_CoorSys_E[x;y][m]_/1(Out1) -> Bus Creator3/44  "Pos_CP_FR_CoorSys_E[x;y][m]"
  Pos_CP_FR_Trailer_CoorSys_E[x;y][m]_/1(Out1) -> Bus Creator3/59  "Pos_CP_FR_Trailer_CoorSys_E[x;y][m]"
  Pos_CP_R2L2_Trailer_CoorSys_E[x;y][m]_/1(Out1) -> Bus Creator3/66  "Pos_CP_R2L2_Trailer_CoorSys_E[x;y][m]"
  Pos_CP_R2L2_CoorSys_E[x;y][m]_/1(Out1) -> Bus Creator3/50  "Pos_CP_R2L2_CoorSys_E[x;y][m]"
  Pos_CP_RL_Trailer_CoorSys_E[x;y][m]_/1(Out1) -> Bus Creator3/61  "Pos_CP_RL_Trailer_CoorSys_E[x;y][m]"
  Pos_CP_RL_CoorSys_E[x;y][m]_/1(Out1) -> Bus Creator3/45  "Pos_CP_RL_CoorSys_E[x;y][m]"
  Pos_CP_RR2_Trailer_CoorSys_E[x;y][m]_/1(Out1) -> Bus Creator3/64  "Pos_CP_RR2_Trailer_CoorSys_E[x;y][m]"
  r_Dyn_Tire[FL;FR;RL;RR][m]_/1(Out1) -> Bus Creator3/6  "r_Dyn_Tire[FL;FR;RL;RR][m]"
  Pos_CP_R2R2_CoorSys_E[x;y][m]_/1(Out1) -> Bus Creator3/52  "Pos_CP_R2R2_CoorSys_E[x;y][m]"
  Pos_CP_RR_CoorSys_E[x;y][m]_/1(Out1) -> Bus Creator3/47  "Pos_CP_RR_CoorSys_E[x;y][m]"
  Const_r_unloaded_Tire_Mean[m]_/1(Out1) -> Bus Creator3/18  "Const_r_unloaded_Tire_Mean[m]"
  Pos_CP_FR2_Trailer_CoorSys_E[x;y][m]_/1(Out1) -> Bus Creator3/60  "Pos_CP_FR2_Trailer_CoorSys_E[x;y][m]"
  Pos_CP_RL2_CoorSys_E[x;y][m]_/1(Out1) -> Bus Creator3/46  "Pos_CP_RL2_CoorSys_E[x;y][m]"
  Pos_CP_FL_CoorSys_E[x;y][m]_/1(Out1) -> Bus Creator3/43  "Pos_CP_FL_CoorSys_E[x;y][m]"
  Pos_CP_FL2_Trailer_CoorSys_E[x;y][m]_/1(Out1) -> Bus Creator3/58  "Pos_CP_FL2_Trailer_CoorSys_E[x;y][m]"
  Pos_CP_RL2_Trailer_CoorSys_E[x;y][m]_/1(Out1) -> Bus Creator3/62  "Pos_CP_RL2_Trailer_CoorSys_E[x;y][m]"
  Pos_CP_R2R_Trailer_CoorSys_E[x;y][m]_/1(Out1) -> Bus Creator3/67  "Pos_CP_R2R_Trailer_CoorSys_E[x;y][m]"
  Pos_CP_R2L_CoorSys_E[x;y][m]_/1(Out1) -> Bus Creator3/49  "Pos_CP_R2L_CoorSys_E[x;y][m]"
  CorneringStiffness[FL;FR;RL;RR][N]_/1(Out1) -> Bus Creator3/8  "CorneringStiffness[FL;FR;RL;RR][N]"
  r_Dyn_Tire[FL;FR;RL;RR][m]/1 -> r_Dyn_Tire[FL;FR;RL;RR][m]_/1(In1)
  Const_r_unloaded_Tire_Mean[m]/1 -> Const_r_unloaded_Tire_Mean[m]_/1(In1)
  Coef_RollingRes[FL;FR;RL;RR][]/1 -> Coef_RollingRes[FL;FR;RL;RR][]_/1(In1)
  Coef_RollingRes_Mean[]/1 -> Coef_RollingRes_Mean[]_/1(In1)
  CorneringStiffness[FL;FR;RL;RR][N]/1 -> CorneringStiffness[FL;FR;RL;RR][N]_/1(In1)
  Pos_CP_FL_CoorSys_E[x;y][m]/1 -> Pos_CP_FL_CoorSys_E[x;y][m]_/1(In1)
  Pos_CP_FR_CoorSys_E[x;y][m]/1 -> Pos_CP_FR_CoorSys_E[x;y][m]_/1(In1)
  Pos_CP_RL_CoorSys_E[x;y][m]/1 -> Pos_CP_RL_CoorSys_E[x;y][m]_/1(In1)
  Pos_CP_RL2_CoorSys_E[x;y][m]/1 -> Pos_CP_RL2_CoorSys_E[x;y][m]_/1(In1)
  Pos_CP_RR_CoorSys_E[x;y][m]/1 -> Pos_CP_RR_CoorSys_E[x;y][m]_/1(In1)
  Pos_CP_RR2_CoorSys_E[x;y][m]/1 -> Pos_CP_RR2_CoorSys_E[x;y][m]_/1(In1)
  Pos_CP_R2L_CoorSys_E[x;y][m]/1 -> Pos_CP_R2L_CoorSys_E[x;y][m]_/1(In1)
  Pos_CP_R2L2_CoorSys_E[x;y][m]/1 -> Pos_CP_R2L2_CoorSys_E[x;y][m]_/1(In1)
  Pos_CP_R2R_CoorSys_E[x;y][m]/1 -> Pos_CP_R2R_CoorSys_E[x;y][m]_/1(In1)
  Pos_CP_R2R2_CoorSys_E[x;y][m]/1 -> Pos_CP_R2R2_CoorSys_E[x;y][m]_/1(In1)
  Pos_CP_FL_Trailer_CoorSys_E[x;y][m]/1 -> Pos_CP_FL_Trailer_CoorSys_E[x;y][m]_/1(In1)
  Pos_CP_FL2_Trailer_CoorSys_E[x;y][m]/1 -> Pos_CP_FL2_Trailer_CoorSys_E[x;y][m]_/1(In1)
  Pos_CP_FR_Trailer_CoorSys_E[x;y][m]/1 -> Pos_CP_FR_Trailer_CoorSys_E[x;y][m]_/1(In1)
  Pos_CP_FR2_Trailer_CoorSys_E[x;y][m]/1 -> Pos_CP_FR2_Trailer_CoorSys_E[x;y][m]_/1(In1)
  Pos_CP_RL_Trailer_CoorSys_E[x;y][m]/1 -> Pos_CP_RL_Trailer_CoorSys_E[x;y][m]_/1(In1)
  Pos_CP_RL2_Trailer_CoorSys_E[x;y][m]/1 -> Pos_CP_RL2_Trailer_CoorSys_E[x;y][m]_/1(In1)
  Pos_CP_RR_Trailer_CoorSys_E[x;y][m]/1 -> Pos_CP_RR_Trailer_CoorSys_E[x;y][m]_/1(In1)
  Pos_CP_RR2_Trailer_CoorSys_E[x;y][m]/1 -> Pos_CP_RR2_Trailer_CoorSys_E[x;y][m]_/1(In1)
  Pos_CP_R2L_Trailer_CoorSys_E[x;y][m]/1 -> Pos_CP_R2L_Trailer_CoorSys_E[x;y][m]_/1(In1)
  Pos_CP_R2L2_Trailer_CoorSys_E[x;y][m]/1 -> Pos_CP_R2L2_Trailer_CoorSys_E[x;y][m]_/1(In1)
  Pos_CP_R2R_Trailer_CoorSys_E[x;y][m]/1 -> Pos_CP_R2R_Trailer_CoorSys_E[x;y][m]_/1(In1)
  Pos_CP_R2R2_Trailer_CoorSys_E[x;y][m]/1 -> Pos_CP_R2R2_Trailer_CoorSys_E[x;y][m]_/1(In1)
  Active_CP_VehDyn_Trailer[]/1 -> Active_CP_VehDyn_Trailer[]_/1(In1)
  AEB[0|1]_/1(Out1) -> Bus Creator3/20  "AEB[0|1]"
  FCW[0|1]_/1(Out1) -> Bus Creator3/21  "FCW[0|1]"
  AEB[0|1]/1 -> AEB[0|1]_/1(In1)
  FCW[0|1]/1 -> FCW[0|1]_/1(In1)
  Gear[]_/1(Out1) -> Bus Creator3/25  "Gear[]"
  s_Preview[m]_/1(Out1) -> Bus Creator3/27  "s_Preview[m]"
  Pos_ClutchPedal[%]_/1(Out1) -> Bus Creator3/24  "Pos_ClutchPedal[%]"
  SelectorLever[-3T|-2P|-1R|0N|1D]_/1(Out1) -> Bus Creator3/26  "SelectorLever[-3T|-2P|-1R|0N|1D]"
  Pos_BrakePedal[%]_/1(Out1) -> Bus Creator3/23  "Pos_BrakePedal[%]"
  t_Preview_vRef_Driver[s]_/1(Out1) -> Bus Creator3/29  "t_Preview_vRef_Driver[s]"
  Angle_SteeringWheel[deg]_/1(Out1) -> Bus Creator3/28  "Angle_SteeringWheel[deg]"
  Pos_AccPedal[%]_/1(Out1) -> Bus Creator3/22  "Pos_AccPedal[%]"
  Pos_AccPedal[%]/1 -> Pos_AccPedal[%]_/1(In1)
  Pos_BrakePedal[%]/1 -> Pos_BrakePedal[%]_/1(In1)
  Pos_ClutchPedal[%]/1 -> Pos_ClutchPedal[%]_/1(In1)
  Gear[]/1 -> Gear[]_/1(In1)
  SelectorLever[-3T|-2P|-1R|0N|1D]/1 -> SelectorLever[-3T|-2P|-1R|0N|1D]_/1(In1)
  s_Preview[m]/1 -> s_Preview[m]_/1(In1)
  Angle_SteeringWheel[deg]/1 -> Angle_SteeringWheel[deg]_/1(In1)
  t_Preview_vRef_Driver[s]/1 -> t_Preview_vRef_Driver[s]_/1(In1)
  a_y_Vehicle_CoG[m|s2]/1 -> a_y_Vehicle_CoG[m|s2]_/1(In1)
  RotationMatrix_V_to_E[1x9]_/1(Out1) -> Bus Creator3/17  "RotationMatrix_V_to_E[1x9]"
  v_x_Vehicle_CoG[km|h]/1 -> v_x_Vehicle_CoG[km|h]_/1(In1)
  Pos_Vehicle_CoorSys_E[x;y;z][m]_/1(Out1) -> Bus Creator3/9  "Pos_Vehicle_CoorSys_E[x;y;z][m]"
  v_y_Vehicle_CoG[km|h]/1 -> v_y_Vehicle_CoG[km|h]_/1(In1)
  RotationMatrix_V_to_E[1x9]/1 -> RotationMatrix_V_to_E[1x9]_/1(In1)
  Angle_Vehicle_CoorSys_E[x;y;z][deg]_/1(Out1) -> Bus Creator3/10  "Angle_Vehicle_CoorSys_E[x;y;z][deg]"
  s_Vehicle[m]_/1(Out1) -> Bus Creator3/11  "s_Vehicle[m]"
  RollRate_Vehicle_CoG[deg|s]/1 -> RollRate_Vehicle_CoG[deg|s]_/1(In1)
  YawRate_Vehicle_CoG[deg|s]_/1(Out1) -> Bus Creator3/15  "YawRate_Vehicle_CoG[deg|s]"
  RollRate_Vehicle_CoG[deg|s]_/1(Out1) -> Bus Creator3/14  "RollRate_Vehicle_CoG[deg|s]"
  s_Vehicle[m]/1 -> s_Vehicle[m]_/1(In1)
  v_y_Vehicle_CoG[km|h]_/1(Out1) -> Bus Creator3/13  "v_y_Vehicle_CoG[km|h]"
  v_x_Vehicle_CoG[km|h]_/1(Out1) -> Bus Creator3/12  "v_x_Vehicle_CoG[km|h]"
  Pos_Vehicle_CoorSys_E[x;y;z][m]/1 -> Pos_Vehicle_CoorSys_E[x;y;z][m]_/1(In1)
  a_y_Vehicle_CoG[m|s2]_/1(Out1) -> Bus Creator3/16  "a_y_Vehicle_CoG[m|s2]"
  YawRate_Vehicle_CoG[deg|s]/1 -> YawRate_Vehicle_CoG[deg|s]_/1(In1)
  Angle_Vehicle_CoorSys_E[x;y;z][deg]/1 -> Angle_Vehicle_CoorSys_E[x;y;z][deg]_/1(In1)
  Mode_Drivetrain[1|2|3|4|5]_/1(Out1) -> Bus Creator3/54  "Mode_Drivetrain[1|2|3|4|5]"
  Sw_MasterBrakeCylinder_Mode[1linear|2physical|3Booster]_/1(Out1) -> Bus Creator3/55  "Sw_MasterBrakeCylinder_Mode[1linear|2physical|3Booster]"
  Mode_Drivetrain[1|2|3|4|5]/1 -> Mode_Drivetrain[1|2|3|4|5]_/1(In1)
  Mode_Transmission[1Manual|2Automatic]_/1(Out1) -> Bus Creator3/53  "Mode_Transmission[1Manual|2Automatic]"
  Mode_Transmission[1Manual|2Automatic]/1 -> Mode_Transmission[1Manual|2Automatic]_/1(In1)
  Sw_MasterBrakeCylinder_Mode[1linear|2physical|3Booster]/1 -> Sw_MasterBrakeCylinder_Mode[1linear|2physical|3Booster]_/1(In1)
  Angle_SteeringWheel_dt_SteeringSystem[deg|s]/1 -> Angle_SteeringWheel_dt_SteeringSystem[deg|s]_/1(In1)
  Angle_SteeringWheel_dt_SteeringSystem[deg|s]_/1(Out1) -> Bus Creator3/4  "Angle_SteeringWheel_dt_SteeringSystem[deg|s]"
  n_Engine_1[rpm]/1 -> n_Engine_1[rpm]_/1(In1)
  n_Engine_1[rpm]_/1(Out1) -> Bus Creator3/32  "n_Engine_1[rpm]"
  Trq_Engine_1[Nm]_/1(Out1) -> Bus Creator3/31  "Trq_Engine_1[Nm]"
  Trq_Engine_1[Nm]/1 -> Trq_Engine_1[Nm]_/1(In1)
  m_TotalVehicle[kg]_/1(Out1) -> Bus Creator3/36  "m_TotalVehicle[kg]"
  m_TotalVehicle[kg]/1 -> m_TotalVehicle[kg]_/1(In1)
  State_StartButton[-2|-1|0|1|2|3]_/1(Out1) -> Bus Creator3/37  "State_StartButton[-2|-1|0|1|2|3]"
  State_StartButton[-2|-1|0|1|2|3]/1 -> State_StartButton[-2|-1|0|1|2|3]_/1(In1)
  ACC_State[1OFF|2Standby|3ON]_/1(Out1) -> Bus Creator3/38  "ACC_State[1OFF|2Standby|3ON]"
  ACC_State[1OFF|2Standby|3ON]/1 -> ACC_State[1OFF|2Standby|3ON]_/1(In1)
  Type_Engine_1[0Unkown|1Other|2Otto|3Diesel|4Electric]/1 -> Type_Engine_1[0Unkown|1Other|2Otto|3Diesel|4Electric]_/1(In1)
  Type_Engine_1[0Unkown|1Other|2Otto|3Diesel|4Electric]_/1(Out1) -> Bus Creator3/30  "Type_Engine_1[0Unkown|1Other|2Otto|3Diesel|4Electric]"
  Type_Engine_2[0Unkown|1Other|2Otto|3Diesel|4Electric]_/1(Out1) -> Bus Creator3/33  "Type_Engine_2[0Unkown|1Other|2Otto|3Diesel|4Electric]"
  Type_Engine_2[0Unkown|1Other|2Otto|3Diesel|4Electric]/1 -> Type_Engine_2[0Unkown|1Other|2Otto|3Diesel|4Electric]_/1(In1)
  Trq_Engine_2[Nm]/1 -> Trq_Engine_2[Nm]_/1(In1)
  Trq_Engine_2[Nm]_/1(Out1) -> Bus Creator3/34  "Trq_Engine_2[Nm]"
  n_Engine_2[rpm]_/1(Out1) -> Bus Creator3/35  "n_Engine_2[rpm]"
  n_Engine_2[rpm]/1 -> n_Engine_2[rpm]_/1(In1)
  Driver_Override_ACC_Active[0Off|1On]/1 -> Driver_Override_ACC_Active[0Off|1On]_/1(In1)
  Driver_Override_ACC_Active[0Off|1On]_/1(Out1) -> Bus Creator3/39  "Driver_Override_ACC_Active[0Off|1On]"
  Driver_Override_ACC_Reason[0NoOverride|1BrakePedal|2AccPedal]/1 -> Driver_Override_ACC_Reason[0NoOverride|1BrakePedal|2AccPedal]_/1(In1)
  Driver_Override_ACC_Reason[0NoOverride|1BrakePedal|2AccPedal]_/1(Out1) -> Bus Creator3/40  "Driver_Override_ACC_Reason[0NoOverride|1BrakePedal|2AccPedal]"
  Slip_x_Wheel[]_/1(Out1) -> Bus Creator3/42  "Slip_x_Wheel[]"
  Slip_x_Wheel[]/1 -> Slip_x_Wheel[]_/1(In1)
  omega_Wheel[rad|s]_/1(Out1) -> Bus Creator3/41  "omega_Wheel[rad|s]"
  omega_Wheel[rad|s]/1 -> omega_Wheel[rad|s]_/1(In1)
